simulink model "LLC_Frequency_Control"  (R2022b)
settings: Solver=VariableStepAuto  StartTime=0.0  StopTime=0.1  RelTol=1e-3
libraries: spsSeriesRLCBranchLib x14, spsMosfetLib x8, spsCurrentMeasurementLib x6, spsVoltageMeasurementLib x4, spsDCVoltageSourceLib x1, spsLinearTransformerLib x1, slpidlib x1, spspowerguiLib x1
settings Model: Creator=20695  LastModifiedBy=20695
settings OptimizationCC: ReuseModelBlockBuffer=on

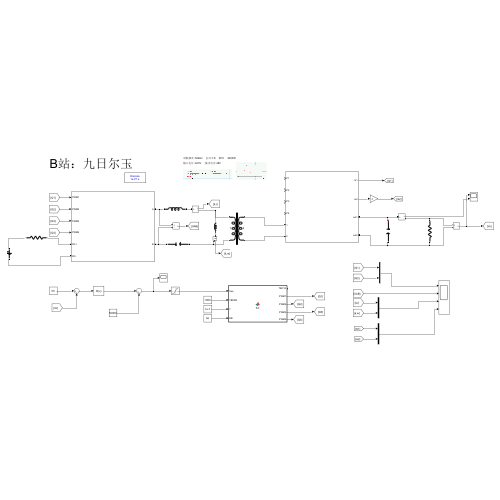
[thumbnail: Simulink's stored preview of the top-level diagram]
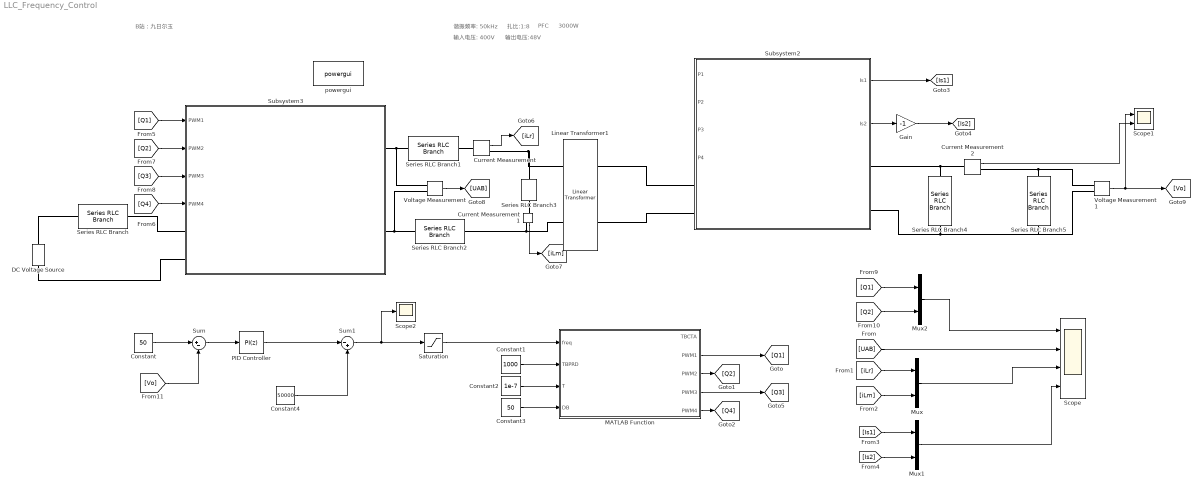
== system LLC_Frequency_Control ==
  note: B站：九日尔玉
  note: 3000W
  note: PFC
  note: 扎比:1:8
  note: 输出电压:48V
  note: 输入电压: 400V
  note: 谐振频率: 50kHz
  Constant : Constant  Value=50
  Constant1 : Constant  Value=1000
  Constant2 : Constant  Value=1e-7
  Constant3 : Constant  Value=50
  Constant4 : Constant  Value=50000
  Current Measurement : spsCurrentMeasurementLib/Current Measurement  PhasorSimulation=off  OutputType=Complex  PSBequivalent=0
  Current Measurement1 : spsCurrentMeasurementLib/Current Measurement  PhasorSimulation=off  OutputType=Complex  PSBequivalent=0
  Current Measurement2 : spsCurrentMeasurementLib/Current Measurement  PhasorSimulation=off  OutputType=Complex  PSBequivalent=0
  DC Voltage Source : spsDCVoltageSourceLib/DC Voltage Source  Amplitude=400  Measurements=None
  Gain : Gain  Gain=-1
  Linear Transformer1 : spsLinearTransformerLib/Linear Transformer  UNITS=SI  NominalPower=[ 3e3 50e3 ]  winding1=[8 0 0]  winding2=[1 0 0]  ThreeWindings=off  winding3=[41.5 1e-4 1e-7]  RmLm=[1e8 0]  Measurements=None  DataType=on
  MATLAB Function : MATLAB Function  TreatAsAtomicUnit=on
  Mux : Mux  Inputs=2
  Mux1 : Mux  Inputs=2
  Mux2 : Mux  Inputs=2
  PID Controller : slpidlib/PID Controller  Controller=PI  Form=Parallel  TimeDomain=Discrete-time  UseExternalTs=off  SampleTime=1e-7  IntegratorMethod=Forward Euler  FilterMethod=Forward Euler  ControllerParametersSource=internal  P=100  I=50000  UseKiTs=off  D=0  N=100  UseFilter=on  TunerSelectOption=Transfer Function Based (PID Tuner App)  InitialConditionSource=internal  InitialConditionForIntegrator=0  InitialConditionForFilter=0  DifferentiatorICPrevScaledInput=0  ExternalReset=none  TrackingMode=off  Kt=1  LimitOutput=off  SatLimitsSource=internal  UpperSaturationLimit=inf  LowerSaturationLimit=-inf  LinearizeAsGain=on  AntiWindupMode=none  Kb=1  LimitIntegrator=off  UpperIntegratorSaturationLimit=inf  LowerIntegratorSaturationLimit=-inf  POutMin=[]  POutMax=[]  IOutMin=[]  IOutMax=[]  DOutMin=[]  DOutMax=[]  NOutMin=[]  NOutMax=[]  SumOutMin=[]  SumOutMax=[]  SaturationOutMin=[]  SaturationOutMax=[]  PParamMin=[]  PParamMax=[]  IParamMin=[]  IParamMax=[]  DParamMin=[]  DParamMax=[]  NParamMin=[]  NParamMax=[]  KbParamMin=[]  KbParamMax=[]  KtParamMin=[]  KtParamMax=[]  KbOutMin=[]  KbOutMax=[]  KtOutMin=[]  KtOutMax=[]  IntegratorOutMin=[]  IntegratorOutMax=[]  FilterOutMin=[]  FilterOutMax=[]  SumI1OutMin=[]  SumI1OutMax=[]  SumI2OutMin=[]  SumI2OutMax=[]  SumI3OutMin=[]  SumI3OutMax=[]  SumI4OutMin=[]  SumI4OutMax=[]  SumDOutMin=[]  SumDOutMax=[]  DifferentiatorOutMin=[]  DifferentiatorOutMax=[]  FilterDiffOutCoefMin=[]  FilterDiffOutCoefMax=[]  ReciprocalOutMin=[]  ReciprocalOutMax=[]  SumDenOutMin=[]  SumDenOutMax=[]  SumNumOutMin=[]  SumNumOutMax=[]  DivideOutMin=[]  DivideOutMax=[]  UdiffTsProdOutMin=[]  UdiffTsProdOutMax=[]  NTsProdOutMin=[]  NTsProdOutMax=[]  UintegralTsProdOutMin=[]  UintegralTsProdOutMax=[]  UngainTsProdOutMin=[]  UngainTsProdOutMax=[]  IntegratorContinuousStateAttributes=''  IntegratorStateMustResolveToSignalObject=off  IntegratorRTWStateStorageClass=Auto  FilterContinuousStateAttributes=''  FilterStateMustResolveToSignalObject=off  FilterRTWStateStorageClass=Auto  ParallelPVariant=InternalParameters  IdealPVariant=Disabled  IVariant=InternalParameters  DVariant=Disabled  IntegratorVariant=Discrete  SatVariant=Disabled  AWVariant=Passthrough  PCopyVariant=Disabled  TRVariant=Disabled  FdbkBlocksVariant=Forward  IdealPFdbkVariant=Disabled  SatFdbkVariant=Disabled  DerivativeFilterVariant=Disabled  NVariant=Disabled  NCopyVariant=Disabled_SignalSpec  FilterICVariant=Disabled  IntegratorICVariant=InternalICs  ExternalResetVariant=Disabled  TRSumVariant=Passthrough  SumFdbkVariant=Disabled  SumVariant=Sum_PI  TsampFilterVariant=InternalTs  TsampNgainVariant=Passthrough  TsampIntegralVariant=Disabled_SignalSpec  ExternalSaturationOutDataTypeStr=Inherit: Same as second input
  Saturation : Saturate  UpperLimit=50000  LowerLimit=35000
  Scope : Scope  NumInputPorts=4
  Scope1 : Scope  NumInputPorts=2
  Scope2 : Scope
  Series RLC Branch : spsSeriesRLCBranchLib/Series RLC Branch  LConnTagsString=__new0  RConnTagsString=__new0  BranchType=R  Resistance=0.0001  Inductance=1e-3  SetiL0=off  InitialCurrent=0  Capacitance=1e-6  Setx0=off  InitialVoltage=0  Measurements=None
  Series RLC Branch1 : spsSeriesRLCBranchLib/Series RLC Branch  LConnTagsString=__new0  RConnTagsString=__new0  BranchType=L  Resistance=0.0001  Inductance=0.078e-3  SetiL0=off  InitialCurrent=0  Capacitance=1e-6  Setx0=off  InitialVoltage=0  Measurements=None
  Series RLC Branch2 : spsSeriesRLCBranchLib/Series RLC Branch  LConnTagsString=__new0  RConnTagsString=__new0  BranchType=C  Resistance=0.0001  Inductance=1e-3  SetiL0=off  InitialCurrent=0  Capacitance=130.508e-9  Setx0=off  InitialVoltage=0  Measurements=None
  Series RLC Branch3 : spsSeriesRLCBranchLib/Series RLC Branch  LConnTagsString=__new0  RConnTagsString=__new0  BranchType=L  Resistance=0.0001  Inductance=0.233e-3  SetiL0=off  InitialCurrent=0  Capacitance=1e-6  Setx0=off  InitialVoltage=0  Measurements=None
  Series RLC Branch4 : spsSeriesRLCBranchLib/Series RLC Branch  LConnTagsString=__new0  RConnTagsString=__new0  BranchType=C  Resistance=1  Inductance=1e-3  SetiL0=off  InitialCurrent=0  Capacitance=2e-3  Setx0=off  InitialVoltage=0  Measurements=None
  Series RLC Branch5 : spsSeriesRLCBranchLib/Series RLC Branch  LConnTagsString=__new0  RConnTagsString=__new0  BranchType=R  Resistance=1  Inductance=1e-3  SetiL0=off  InitialCurrent=0  Capacitance=2e-3  Setx0=off  InitialVoltage=0  Measurements=None
  Subsystem2 : Subsystem  mask{C=0}
      mask DialogControl ParameterGroupVar Prompt: 参数
  Subsystem3 : Subsystem  mask{C=330e-12}
      mask prompts: C "寄生电容大小"
      mask DialogControl ParameterGroupVar Prompt: 参数
  Sum : Sum  Inputs=|+-
  Sum1 : Sum  Inputs=|-+
  Voltage Measurement : spsVoltageMeasurementLib/Voltage Measurement  PhasorSimulation=off  OutputType=Complex  PSBequivalent=0
  Voltage Measurement1 : spsVoltageMeasurementLib/Voltage Measurement  PhasorSimulation=off  OutputType=Complex  PSBequivalent=0
  powergui : spspowerguiLib/powergui  Priority=1  SimulationMode=Discrete  SampleTime=1e-7  frequency=60  Iterations=50  frequencyindice=0  Pbase=100e6  ErrMax=1e-4  UnitsV=kV  UnitsW=MW  buscounter=0  FunctionMessages=off  echomessages=off  EnableUseOfTLC=off  CurrentSourceSwitches=off  DisableSnubberDevices=off  DisableRonSwitches=off  DisableVfSwitches=off  DisplayEquations=off  AutomaticDiscreteSolvers=off  SolverType=Tustin/Backward Euler (TBE)  Interpol=off  ExternalGateDelay=off  methode=off  Ts=100  x0status=blocks  SPID=on  SwTol=0  HookPort=off  NonlinearTolerance=1e-4  nMaxIteration=100  ContinueOnMaxIteration=off  RestoreLinks=warning  ResistiveCurrentMeasurement=off  Frange=[0:2:500]  Ylog=off  Xlog=on  ShowGrid=off  save=off  variable=ZData  structure=0  ZoomFFT=off  StartTime=0.0  cycles=1  DisplayStyle=1  fundamental=60  FreqAxis=off  MaxFrequency=1000  frequencyindicesteady=1  RmsSteady=1  display=off
  wires:
  [UAB] -> Scope/2
  [iLr] -> Mux/1
  [iLm] -> Mux/2
  Mux/1 -> Scope/3
  Subsystem2/2(Is2) -> Gain/1
  Gain/1 -> [Is2]
  Subsystem2/1(Is1) -> [Is1]
  [Is1] -> Mux1/1
  [Is2] -> Mux1/2
  Mux1/1 -> Scope/4
  [Q1] -> Mux2/1
  [Q2] -> Mux2/2
  Mux2/1 -> Scope/1
  [Q1] -> Subsystem3/1(PWM1)
  [Q2] -> Subsystem3/2(PWM2)
  [Q3] -> Subsystem3/3(PWM3)
  [Q4] -> Subsystem3/4(PWM4)
  Current Measurement/1 -> [iLr]
  Current Measurement1/1 -> [iLm]
  Voltage Measurement/1 -> [UAB]
  Voltage Measurement1/1 -> [Vo], Scope1/1
  Current Measurement2/1 -> Scope1/2
  Constant3/1 -> MATLAB Function/4(DB)
  Constant1/1 -> MATLAB Function/2(TBPRD)
  Constant2/1 -> MATLAB Function/3(T)
  MATLAB Function/2(PWM1) -> [Q1]
  MATLAB Function/5(PWM4) -> [Q4]
  MATLAB Function/3(PWM2) -> [Q2]
  MATLAB Function/4(PWM3) -> [Q3]
  Constant/1 -> Sum/1
  [Vo] -> Sum/2
  Sum/1 -> PID Controller/1
  PID Controller/1 -> Sum1/1
  Constant4/1 -> Sum1/2
  Sum1/1 -> Saturation/1, Scope2/1
  Saturation/1 -> MATLAB Function/1(freq)
  connections:
  Series RLC Branch/RConn1 -- Subsystem3/LConn1
  DC Voltage Source/RConn1 -- Series RLC Branch/LConn1
  DC Voltage Source/LConn1 -- Subsystem3/LConn2
  Current Measurement/LConn1 -- Series RLC Branch1/RConn1
  Current Measurement1/LConn1 -- Series RLC Branch3/RConn1
  Current Measurement/RConn1 -- Linear Transformer1/LConn1 -- Series RLC Branch3/LConn1
  Series RLC Branch2/RConn1 -- Linear Transformer1/LConn2 -- Current Measurement1/RConn1
  Subsystem3/RConn1 -- Voltage Measurement/LConn1 -- Series RLC Branch1/LConn1
  Subsystem3/RConn2 -- Voltage Measurement/LConn2 -- Series RLC Branch2/LConn1
  Linear Transformer1/RConn1 -- Subsystem2/LConn1
  Linear Transformer1/RConn2 -- Subsystem2/LConn2
  Subsystem2/RConn1 -- Current Measurement2/LConn1 -- Series RLC Branch4/LConn1
  Subsystem2/RConn2 -- Voltage Measurement1/LConn2 -- Series RLC Branch5/RConn1 -- Series RLC Branch4/RConn1
  Current Measurement2/RConn1 -- Voltage Measurement1/LConn1 -- Series RLC Branch5/LConn1

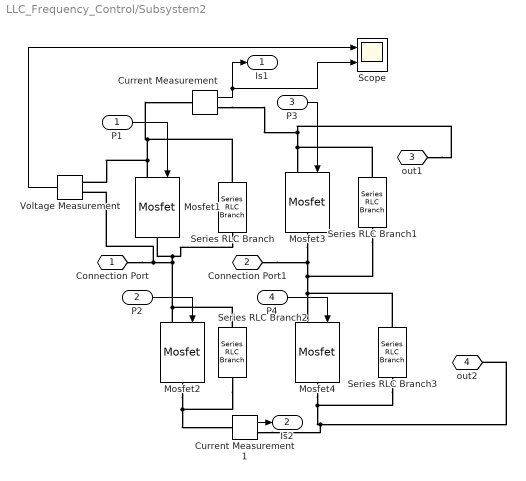
== system LLC_Frequency_Control/Subsystem2 ==
  P1 : Inport
  P2 : Inport  Port=2
  P3 : Inport  Port=3
  P4 : Inport  Port=4
  Current Measurement : spsCurrentMeasurementLib/Current Measurement  PhasorSimulation=off  OutputType=Complex  PSBequivalent=0
  Current Measurement1 : spsCurrentMeasurementLib/Current Measurement  PhasorSimulation=off  OutputType=Complex  PSBequivalent=0
  Mosfet{1..4} (4 alike) : spsMosfetLib/Mosfet  Ron=0.1  Lon=0  Rd=0.01  Vfd=1.5  IC=0  Rs=1e5  Cs=inf  Measurements=off
  Scope : Scope  NumInputPorts=2
  Series RLC Branch{,1..3} (4 alike) : spsSeriesRLCBranchLib/Series RLC Branch  LConnTagsString=__new0  RConnTagsString=__new0  BranchType=C  Resistance=1  Inductance=1e-3  SetiL0=off  InitialCurrent=0  Capacitance=C  Setx0=off  InitialVoltage=0  Measurements=None
  Voltage Measurement : spsVoltageMeasurementLib/Voltage Measurement  PhasorSimulation=off  OutputType=Complex  PSBequivalent=0
  Connection Port : PMIOPort  Side=Left
  Connection Port1 : PMIOPort  Port=2  Side=Left
  out1 : PMIOPort  Port=3  Side=Right
  out2 : PMIOPort  Port=4  Side=Right
  Is1 : Outport
  Is2 : Outport  Port=2
  wires:
  P1/1 -> Mosfet1/1
  P2/1 -> Mosfet2/1
  P3/1 -> Mosfet3/1
  P4/1 -> Mosfet4/1
  Current Measurement/1 -> Is1/1, Scope/2
  Current Measurement1/1 -> Is2/1
  Voltage Measurement/1 -> Scope/1
  connections:
  Series RLC Branch2/LConn1 -- Mosfet2/LConn1 -- Voltage Measurement/LConn2 -- Connection Port/RConn1 -- Series RLC Branch/RConn1 -- Mosfet1/RConn1
  Mosfet3/RConn1 -- Connection Port1/RConn1 -- Series RLC Branch1/RConn1 -- Series RLC Branch3/LConn1 -- Mosfet4/LConn1
  out1/RConn1 -- Current Measurement/RConn1 -- Series RLC Branch1/LConn1 -- Mosfet3/LConn1
  out2/RConn1 -- Series RLC Branch3/RConn1 -- Mosfet4/RConn1 -- Current Measurement1/RConn1
  Mosfet1/LConn1 -- Voltage Measurement/LConn1 -- Current Measurement/LConn1 -- Series RLC Branch/LConn1
  Mosfet2/RConn1 -- Series RLC Branch2/RConn1 -- Current Measurement1/LConn1

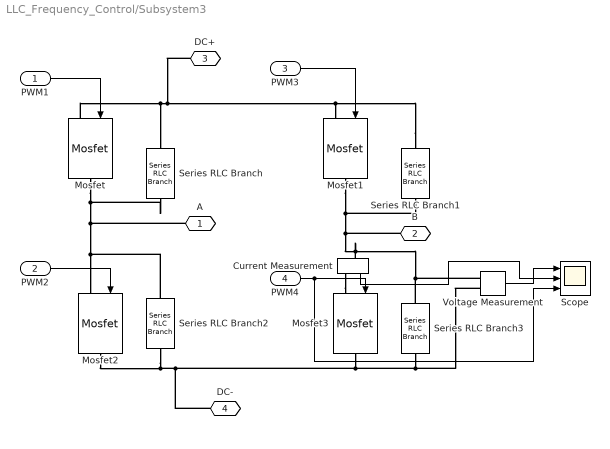
== system LLC_Frequency_Control/Subsystem3 ==
  PWM1 : Inport
  PWM2 : Inport  Port=2
  PWM3 : Inport  Port=3
  PWM4 : Inport  Port=4
  Current Measurement : spsCurrentMeasurementLib/Current Measurement  PhasorSimulation=off  OutputType=Complex  PSBequivalent=0
  Mosfet{,1..3} (4 alike) : spsMosfetLib/Mosfet  Ron=0.1  Lon=0  Rd=0.01  Vfd=0  IC=0  Rs=1e5  Cs=inf  Measurements=off
  Scope : Scope  NumInputPorts=3
  Series RLC Branch{,1..3} (4 alike) : spsSeriesRLCBranchLib/Series RLC Branch  LConnTagsString=__new0  RConnTagsString=__new0  BranchType=C  Resistance=1  Inductance=1e-3  SetiL0=off  InitialCurrent=0  Capacitance=C  Setx0=off  InitialVoltage=0  Measurements=None
  Voltage Measurement : spsVoltageMeasurementLib/Voltage Measurement  PhasorSimulation=off  OutputType=Complex  PSBequivalent=0
  A : PMIOPort  Side=Right
  B : PMIOPort  Port=2  Side=Right
  DC+ : PMIOPort  Port=3  Side=Left
  DC- : PMIOPort  Port=4  Side=Left
  wires:
  PWM1/1 -> Mosfet/1
  PWM4/1 -> Scope/3, Mosfet3/1
  PWM3/1 -> Mosfet1/1
  PWM2/1 -> Mosfet2/1
  Current Measurement/1 -> Scope/2
  Voltage Measurement/1 -> Scope/1
  connections:
  Series RLC Branch3/LConn1 -- Series RLC Branch1/RConn1 -- Mosfet1/RConn1 -- B/RConn1 -- Current Measurement/LConn1 -- Voltage Measurement/LConn1
  Series RLC Branch1/LConn1 -- Mosfet1/LConn1 -- Mosfet/LConn1 -- Series RLC Branch/LConn1 -- DC+/RConn1
  Series RLC Branch/RConn1 -- Mosfet/RConn1 -- Series RLC Branch2/LConn1 -- Mosfet2/LConn1 -- A/RConn1
  Mosfet2/RConn1 -- Series RLC Branch2/RConn1 -- Voltage Measurement/LConn2 -- Series RLC Branch3/RConn1 -- Mosfet3/RConn1 -- DC-/RConn1
  Current Measurement/RConn1 -- Mosfet3/LConn1

== matlab function LLC_Frequency_Control/MATLAB Function ==
  data: freq input; TBCTA output; TBPRD input; T input; DB input; PWM1 output; PWM2 output; PWM3 output; PWM4 output
function [TBCTA,PWM1,PWM2,PWM3,PWM4]  = fcn(freq,TBPRD,T,DB)
persistent out1;
if isempty(out1)
    out1=0;
end
persistent flag;
if isempty(flag)
    flag=0;
end

persistent P1;
if isempty(P1)
    P1=0;
end
persistent P2;
if isempty(P2)
    P2=0;
end

Ts = 1/freq;
if flag == 0
    out1 = out1 + TBPRD/(Ts/2/T);%增计算
    if out1 > 950
        P1 = 0;
    end

else
    out1 = out1 -  TBPRD/(Ts/2/T);%减计算
    if out1 < 50
        P2 = 0;
    end
end
if out1 > TBPRD
   out1 = TBPRD;
   flag = 1;
   P1 = 0;
   P2 = 1;
end
if out1 < 0
   out1 = 0;
   flag = 0;
   P1 = 1;
   P2 = 0;
end
PWM1 = P1;
PWM4 = P1;
PWM3 = P2;
PWM2 = P2;
TBCTA = out1;
